simulink model "xfm_reference"  (R2025b)
settings: Solver=ode4  StartTime=0.0  StopTime=20  FixedStep=xfm_cfg.dt  RelTol=1e-3
undefined symbols (not defined in the file or in its folder): xfm_cfg
libraries: aerolibprivatev1p5 x1, aerolibatmos2 x1
settings Model: Creator=schultz  LastModifiedBy=schultz
settings DataIOCC: SignalLogging=off

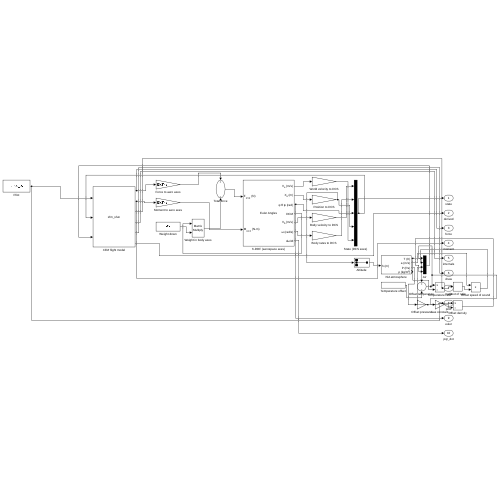
[thumbnail: Simulink's stored preview of the top-level diagram]
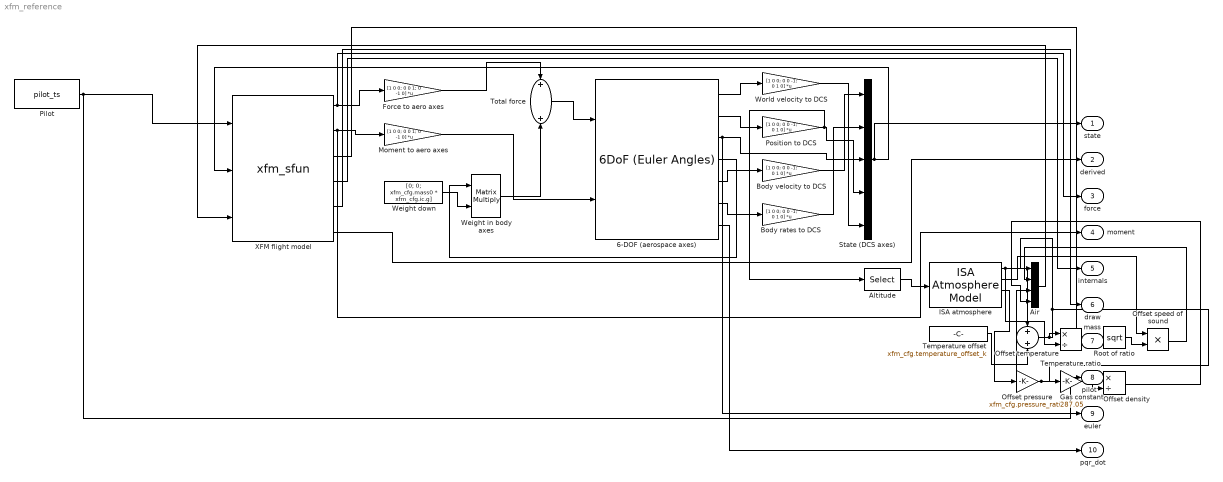
== system xfm_reference ==
  6-DOF (aerospace axes) : aerolibprivatev1p5/6DoF (Euler Angles)  xme_0=xfm_cfg.ic.xe0  Vm_0=xfm_cfg.ic.vb0_aero  eul_0=xfm_cfg.ic.eul0  pm_0=xfm_cfg.ic.pqr0  Mass=xfm_cfg.mass0  Inertia=xfm_cfg.inertia_aero
  Air : Mux
  Altitude : Selector  InputPortWidth=3  IndexOptions=Index vector (dialog)  Indices=2  OutputSizes=1
  Body rates to DCS : Gain  Gain=[1 0 0; 0 0 -1; 0 1 0]  Multiplication=Matrix(K*u)
  Body velocity to DCS : Gain  Gain=[1 0 0; 0 0 -1; 0 1 0]  Multiplication=Matrix(K*u)
  Force to aero axes : Gain  Gain=[1 0 0; 0 0 1; 0 -1 0]  Multiplication=Matrix(K*u)
  Gas constant : Gain  Gain=287.05
  ISA atmosphere : aerolibatmos2/ISA Atmosphere Model  useExtended=off  action=None  custom=off  viscosityOut=off  g=9.80665  gamma=1.4  R=287.0531  L=0.0065  h_trop=11000  h_strat=20000  rho0=1.225  P0=101325  T0=288.15  h0=0  S=110.4  Tref=273.15  muref=1.716e-5
  Moment to aero axes : Gain  Gain=[1 0 0; 0 0 1; 0 -1 0]  Multiplication=Matrix(K*u)
  Offset density : Product  Inputs=*/
  Offset pressure : Gain  Gain=xfm_cfg.pressure_ratio
  Offset speed of sound : Product  Inputs=**
  Offset temperature : Sum
  Pilot : FromWorkspace  VariableName=pilot_ts  SampleTime=xfm_cfg.dt  Interpolate=off  OutputAfterFinalValue=Holding final value
  Position to DCS : Gain  Gain=[1 0 0; 0 0 -1; 0 1 0]  Multiplication=Matrix(K*u)
  Root of ratio : Math  Operator=sqrt
  State (DCS axes) : Mux  Inputs=5
  Temperature offset : Constant  Value=xfm_cfg.temperature_offset_k
  Temperature ratio : Product  Inputs=*/
  Total force : Sum
  Weight down : Constant  Value=[0; 0; xfm_cfg.mass0 * xfm_cfg.ic.g]
  Weight in body axes : Product  Multiplication=Matrix(*)
  World velocity to DCS : Gain  Gain=[1 0 0; 0 0 -1; 0 1 0]  Multiplication=Matrix(K*u)
  XFM flight model : S-Function  FunctionName=xfm_sfun  Parameters=xfm_cfg.library, xfm_cfg.config_dir, xfm_cfg.run_dir, xfm_cfg.settings, xfm_cfg.dt, xfm_cfg.engines  SFunctionDeploymentMode=off  EnableBusSupport=off
  state : Outport
  derived : Outport  Port=2
  force : Outport  Port=3
  moment : Outport  Port=4
  internals : Outport  Port=5
  draw : Outport  Port=6
  mass : Outport  Port=7
  pilot : Outport  Port=8
  euler : Outport  Port=9
  pqr_dot : Outport  Port=10
  wires:
  Pilot/1 -> XFM flight model/1, pilot/1
  XFM flight model/1 -> Force to aero axes/1, force/1
  XFM flight model/2 -> Moment to aero axes/1, moment/1
  Weight down/1 -> Weight in body axes/2
  6-DOF (aerospace axes)/4 -> Weight in body axes/1
  Force to aero axes/1 -> Total force/1
  Weight in body axes/1 -> Total force/2
  Total force/1 -> 6-DOF (aerospace axes)/1
  Moment to aero axes/1 -> 6-DOF (aerospace axes)/2
  6-DOF (aerospace axes)/1 -> World velocity to DCS/1
  6-DOF (aerospace axes)/2 -> Position to DCS/1
  6-DOF (aerospace axes)/5 -> Body velocity to DCS/1
  6-DOF (aerospace axes)/6 -> Body rates to DCS/1
  Body velocity to DCS/1 -> State (DCS axes)/1
  Body rates to DCS/1 -> State (DCS axes)/2
  6-DOF (aerospace axes)/3 -> State (DCS axes)/3, euler/1
  Position to DCS/1 -> State (DCS axes)/4, Altitude/1
  World velocity to DCS/1 -> State (DCS axes)/5
  State (DCS axes)/1 -> XFM flight model/2, state/1
  Altitude/1 -> ISA atmosphere/1
  ISA atmosphere/3 -> Offset pressure/1
  ISA atmosphere/1 -> Offset temperature/1, Temperature ratio/2
  Temperature offset/1 -> Offset temperature/2
  Offset temperature/1 -> Air/1, Gas constant/1, Temperature ratio/1
  Temperature ratio/1 -> Root of ratio/1
  ISA atmosphere/2 -> Offset speed of sound/1
  Root of ratio/1 -> Offset speed of sound/2
  Offset pressure/1 -> Offset density/1, Air/3
  Gas constant/1 -> Offset density/2
  Offset speed of sound/1 -> Air/2
  Offset density/1 -> Air/4
  Air/1 -> XFM flight model/3
  XFM flight model/6 -> derived/1
  XFM flight model/4 -> internals/1
  XFM flight model/5 -> draw/1
  XFM flight model/3 -> mass/1
  6-DOF (aerospace axes)/7 -> pqr_dot/1
